simulink model "ProyectoSimulinkV1"  (R2025a)
settings: Solver=FixedStepDiscrete  StartTime=0.0  StopTime=inf  FixedStep=0.01  RelTol=1e-3  EnableMultiTasking=on
libraries: simulink_extras x6, arduinolib x6, arduinosensorlib x2
settings Model: SILPILModeSetting=veronly  ExtModeTrigDuration=2  Creator=adria  LastModifiedBy=adria
settings SolverCC: AutoInsertRateTranBlk=on
settings OptimizationCC: EnhancedBackFolding=on  PassReuseOutputArgsAs=Individual arguments  ZeroExternalMemoryAtStartup=off  ZeroInternalMemoryAtStartup=off  MaxStackSize=64  OptimizeBlockOrder=speed  DifferentSizesBufferReuse=on  OptimizationCustomize=off  EfficientTunableParamExpr=on
settings DebuggingCC: ParameterTunabilityLossMsg=error
settings HardwareCC: ProdBitPerPointer=32.0  ProdBitPerSizeT=32.0  ProdBitPerPtrDiffT=32.0  ProdLargestAtomicInteger=Long  ProdLargestAtomicFloat=Double  ProdWordSize=32.0  ProdHWDeviceType=ARM Compatible->ARM Cortex
settings SFSimCC: MATLABDynamicMemAlloc=off
settings RTWCC: SystemTargetFile=ert.tlc  HardwareBoard=ESP32-WROOM (Arduino Compatible)  TLCOptions="-aInlineSetEventsForThisBaseRateFcn=TLC_FALSE -aSuppressMultiTaskScheduler=TLC_FALSE  -aRateBasedStepFcn=0"  TemplateMakefile=ert_default_tmf  Toolchain=ESP32  BuildConfiguration=Faster Runs  Description=Embedded Coder
settings CodeAppCC: ForceParamTrailComments=on  IgnoreCustomStorageClasses=off  OperatorAnnotations=on  SimulinkDataObjDesc=on  SFDataObjDesc=on  InsertBlockDesc=on
settings ERTTargetCC: ExtModeTransport=3.0  ExtModeAutomaticAllocSize=off  ExtModeStaticAllocSize=65536.0  InlinedParameterPlacement=Hierarchical  SupportContinuousTime=on  SupportVariableSizeSignals=on

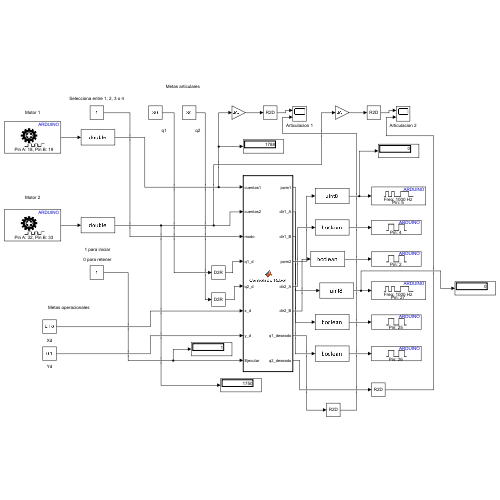
[thumbnail: Simulink's stored preview of the top-level diagram]
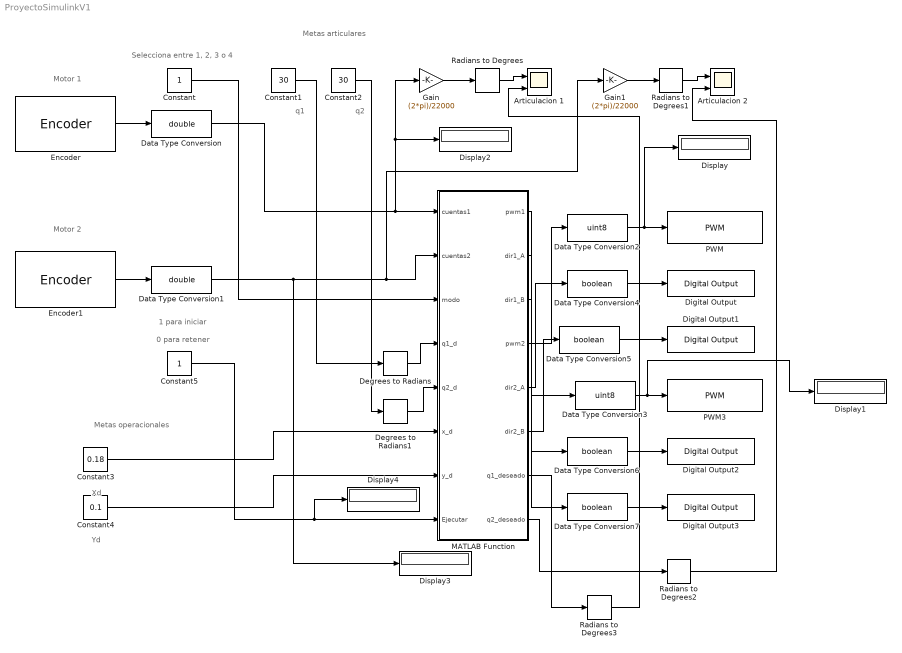
== system ProyectoSimulinkV1 ==
  note: 0 para retener
  note: 1 para iniciar
  note: Yd
  note: Xd
  note: Metas operacionales
  note: q2
  note: q1
  note: Metas articulares
  note: Selecciona entre 1, 2, 3 o 4
  note: Motor 2
  note: Motor 1
  Articulacion 1 : Scope  NumInputPorts=2
      settings: ActiveDisplayYMinimum=-116.05295454545454  ActiveDisplayYMaximum=234.64022727272726
  Articulacion 2 : Scope  NumInputPorts=2
      settings: ActiveDisplayYMinimum=-145.81022727272727  ActiveDisplayYMaximum=203.65568181818182
  Constant : Constant  OutDataTypeStr=double
  Constant1 : Constant  Value=30
  Constant2 : Constant  Value=30
  Constant3 : Constant  Value=0.18  OutDataTypeStr=double
  Constant4 : Constant  Value=0.1  OutDataTypeStr=double
  Constant5 : Constant  OutDataTypeStr=double
  Data Type Conversion : DataTypeConversion  OutDataTypeStr=double  SaturateOnIntegerOverflow=off  RndMeth=Floor
  Data Type Conversion1 : DataTypeConversion  OutDataTypeStr=double  SaturateOnIntegerOverflow=off  RndMeth=Floor
  Data Type Conversion2 : DataTypeConversion  OutDataTypeStr=uint8  SaturateOnIntegerOverflow=off  RndMeth=Floor
  Data Type Conversion3 : DataTypeConversion  OutDataTypeStr=uint8  SaturateOnIntegerOverflow=off  RndMeth=Floor
  Data Type Conversion{4..7} (4 alike) : DataTypeConversion  OutDataTypeStr=boolean  SaturateOnIntegerOverflow=off  RndMeth=Floor
  Degrees to Radians : simulink_extras/Transformations/Degrees to Radians
  Degrees to Radians1 : simulink_extras/Transformations/Degrees to Radians
  Digital Output : arduinolib/Digital Output  pinNumber=4  Direction=output  blockPlatform=arduino
  Digital Output1 : arduinolib/Digital Output  pinNumber=2  Direction=output  blockPlatform=arduino
  Digital Output2 : arduinolib/Digital Output  pinNumber=25  Direction=output  blockPlatform=arduino
  Digital Output3 : arduinolib/Digital Output  pinNumber=26  Direction=output  blockPlatform=arduino
  Display{,1..4} (5 alike) : Display
  Encoder : arduinosensorlib/Encoder  InputA=18  InputB=19  Mode=No reset  SampleTime=0.01
  Encoder1 : arduinosensorlib/Encoder  InputA=32  InputB=33  Mode=No reset  SampleTime=0.01
  Gain : Gain  Gain=(2*pi)/22000
  Gain1 : Gain  Gain=(2*pi)/22000
  MATLAB Function : MATLAB Function  TreatAsAtomicUnit=on
  PWM : arduinolib/PWM  pinNumber=5  frequencyType=Specify  desiredFrequency=1000  achievableFrequency=1000
  PWM3 : arduinolib/PWM  pinNumber=27  frequencyType=Specify  desiredFrequency=1000  achievableFrequency=1000
  Radians to Degrees{,1..3} (4 alike) : simulink_extras/Transformations/Radians to Degrees
  wires:
  Encoder/1 -> Data Type Conversion/1
  Encoder1/1 -> Data Type Conversion1/1
  Degrees to Radians/1 -> MATLAB Function/4(q1_d)
  Degrees to Radians1/1 -> MATLAB Function/5(q2_d)
  Constant1/1 -> Degrees to Radians/1
  Constant2/1 -> Degrees to Radians1/1
  Constant/1 -> MATLAB Function/3(modo)
  Constant3/1 -> MATLAB Function/6(x_d)
  Constant4/1 -> MATLAB Function/7(y_d)
  Data Type Conversion/1 -> Gain/1, Display2/1, MATLAB Function/1(cuentas1)
  Data Type Conversion1/1 -> Display3/1, Gain1/1, MATLAB Function/2(cuentas2)
  Constant5/1 -> MATLAB Function/8(Ejecutar), Display4/1
  Data Type Conversion2/1 -> Display/1, PWM/1
  Data Type Conversion3/1 -> Display1/1, PWM3/1
  Data Type Conversion5/1 -> Digital Output1/1
  Data Type Conversion4/1 -> Digital Output/1
  Data Type Conversion6/1 -> Digital Output2/1
  Data Type Conversion7/1 -> Digital Output3/1
  MATLAB Function/3(dir1_B) -> Data Type Conversion7/1
  MATLAB Function/2(dir1_A) -> Data Type Conversion6/1
  MATLAB Function/1(pwm1) -> Data Type Conversion3/1
  MATLAB Function/4(pwm2) -> Data Type Conversion2/1
  MATLAB Function/5(dir2_A) -> Data Type Conversion4/1
  MATLAB Function/6(dir2_B) -> Data Type Conversion5/1
  Radians to Degrees/1 -> Articulacion 1/1
  Gain/1 -> Radians to Degrees/1
  Gain1/1 -> Radians to Degrees1/1
  Radians to Degrees1/1 -> Articulacion 2/1
  Radians to Degrees2/1 -> Articulacion 2/2
  Radians to Degrees3/1 -> Articulacion 1/2
  MATLAB Function/7(q1_deseado) -> Radians to Degrees3/1
  MATLAB Function/8(q2_deseado) -> Radians to Degrees2/1

== matlab function ProyectoSimulinkV1/MATLAB Function ==
  data: cuentas1 input; pwm1 output; cuentas2 input; modo input; q1_d input; q2_d input; x_d input; y_d input; dir1_A output; dir1_B output; pwm2 output; dir2_A output; dir2_B output; Ejecutar input; q1_deseado output; q2_deseado output
function [pwm1, dir1_A, dir1_B, pwm2, dir2_A, dir2_B, q1_deseado, q2_deseado] = ControladorRobot(cuentas1, cuentas2, modo, q1_d, q2_d, x_d, y_d, Ejecutar)

    % =========================================================================
    % DECLARACIÓN PERSISTENTE
    % =========================================================================
    persistent q_ant meta_q1 meta_q2 meta_x meta_y;
    if isempty(q_ant)
        q_ant = [0; 0];
        meta_q1 = 0; meta_q2 = 0;
        meta_x = 0.315; meta_y = 0; 
    end

    % =========================================================================
    % PARAMETROS ELECTROMECÁNICOS Y FÍSICOS REALES 
    % =========================================================================
    PPR = 22000; R = 8.5; Kt = 0.012; Ke = 0.012; V_max = 12.27; 
    m1 = 0.181; m2 = 0.064; a1 = 0.160; a2 = 0.155; a1c = 0.040; a2c = 0.049; 
    dt = 0.01;   

    if Ejecutar == 1
        meta_q1 = q1_d; meta_q2 = q2_d;
        meta_x = x_d; meta_y = y_d;
    end
    
    % =========================================================================
    % A. LECTURA DE SENSORES Y VELOCIDAD
    % =========================================================================
    q1 = (double(cuentas1) / PPR) * 2 * pi;
    q2 = (double(cuentas2) / PPR) * 2 * pi;
    q_act = [q1; q2];
    qp_act = (q_act - q_ant) / dt; 
    q_ant = q_act;
    
    % =========================================================================
    % B. GRAVEDAD DINÁMICA ANALÍTICA
    % =========================================================================
    g_grav = 0;
    if (modo == 3) || (modo == 4), g_grav = 9.81; end
    
    t2 = cos(q_act(1)); t5 = q_act(1) + q_act(2); t7 = cos(t5);
    gq = [g_grav * m2 * (a1 * t2 + a2c * t7) + a1c * g_grav * m1 * t2 ; 
          a2c * g_grav * m2 * t7];
          
    % =========================================================================
    % CALCULO DE REFERENCIA (Cinemática Inversa Corregida)
    % =========================================================================
    if (modo == 1) || (modo == 3)
        q1_deseado = meta_q1; q2_deseado = meta_q2;
    else
        D = (meta_x^2 + meta_y^2 - a1^2 - a2^2) / (2 * a1 * a2);
        if abs(D) > 1, D = sign(D) * 1; end
        % Invertimos el signo para configuración de codo abajo
        q2_deseado = -atan2(sqrt(1 - D^2), D); 
        q1_deseado = atan2(meta_y, meta_x) - atan2(a2 * sin(q2_deseado), a1 + a2 * cos(q2_deseado));
        
        q1_deseado = mod(q1_deseado + pi, 2*pi) - pi;
        q2_deseado = mod(q2_deseado + pi, 2*pi) - pi;
    end

    % =========================================================================
    % C. LEYES DE CONTROL
    % =========================================================================
    if (modo == 1) || (modo == 3)
        % Articular: Estable
        Kp = diag([0.09, 0.16]); Kd = diag([0.04, 0.03]); 
        e = [meta_q1; meta_q2] - q_act;
        for i = 1:2
            if abs(e(i)) < 0.055, e(i) = 0; qp_act(i) = 0; end
        end
        tau = (Kp * e) - (Kd * qp_act) + gq;
    else
        % --- CONTROL OPERACIONAL: Ganancias estilo Articular (Sintonización Segura) ---
        % Subimos Kp_op para asegurar torque de arranque y Kd_op para estabilidad
        Kp_op = diag([4, 3.5]); 
        Kd_op = diag([0.6, 0.6]);
        
        x_act = [ a1*cos(q_act(1)) + a2*cos(q_act(1)+q_act(2)) ;
                  a1*sin(q_act(1)) + a2*sin(q_act(1)+q_act(2)) ];
                  
        J = [ -a1*sin(q_act(1)) - a2*sin(q_act(1)+q_act(2)), -a2*sin(q_act(1)+q_act(2)) ;
               a1*cos(q_act(1)) + a2*cos(q_act(1)+q_act(2)),  a2*cos(q_act(1)+q_act(2)) ];
               
        e_x = [meta_x; meta_y] - x_act;
        
        % Zona muerta: dejamos una tolerancia de 1.5 cm para evitar chillidos
        if norm(e_x) < 0.015
            e_x = [0; 0]; qp_act = [0; 0];
        end
        
        % Ley de control estrictamente como la de tu presentación:
        tau = J' * (Kp_op * e_x - Kd_op * (J * qp_act)) + gq;
    end

    % =========================================================================
    % D. ACTUACIÓN FÍSICA
    % =========================================================================
    V_req1 = (tau(1) / Kt) * R + (Ke * qp_act(1));
    pwm1 = min(max(abs(V_req1) / V_max, 0), 1) * 255; 
    dir1_A = V_req1 > 0; dir1_B = ~dir1_A;
    V_req2 = (tau(2) / Kt) * R + (Ke * qp_act(2));
    pwm2 = min(max(abs(V_req2) / V_max, 0), 1) * 255;
    dir2_A = V_req2 > 0; dir2_B = ~dir2_A;
end
